simulink model "StampFly_KF400"  (R2026b)
settings: Solver=FixedStepDiscrete  StopTime=inf  FixedStep=Official.Step
PostLoadFcn:
  | run(fullfile(fileparts(get_param('StampFly_KF400','FileName')),'config','startup.m'));
InitFcn:
  | init_kf_flight;
undefined symbols (not defined in the file): AltitudeKF, Bottom, Discrete, Official, Time
libraries: slpidlib x7, simulink x4, ctrlSharedLib x1, mspfiltlib x1
(part 1 of 4)
settings Model: SILPILModeSetting=veronly  Creator=tyasukaw  LastModifiedBy=tyasukaw
settings SolverCC: AutoInsertRateTranBlk=on
settings OptimizationCC: DifferentSizesBufferReuse=on  EfficientTunableParamExpr=on  EnhancedBackFolding=on  MaxStackSize=64  OptimizationCustomize=off  OptimizeBlockOrder=speed  PassReuseOutputArgsAs=Individual arguments  RemoveInternalMemoryZeroInit=on  RemoveRootLevelIOMemoryZeroInit=on
settings DebuggingCC: ParameterTunabilityLossMsg=error
settings HardwareCC: ProdHWDeviceType=ARM Compatible->ARM Cortex  ProdLargestAtomicFloat=Double  ProdLargestAtomicInteger=Long
settings SFSimCC: MATLABDynamicMemAlloc=off
settings RTWCC: BuildConfiguration=Faster Runs  DataTypeReplacement=CDataTypesFixedWidth  Description=Embedded Coder  HardwareBoard=ESP32-S3 Series (Arduino Compatible)  SystemTargetFile=ert.tlc  TLCOptions="-aInlineSetEventsForThisBaseRateFcn=TLC_FALSE -aSuppressMultiTaskScheduler=TLC_FALSE  -aRateBasedStepFcn=0"  TemplateMakefile=ert_default_tmf  Toolchain=ESP32
settings CodeAppCC: ForceParamTrailComments=on  IgnoreCustomStorageClasses=off  InsertBlockDesc=on  OperatorAnnotations=on  SFDataObjDesc=on  SimulinkDataObjDesc=on
settings ERTTargetCC: CombineSignalStateStructs=on  ExtModeAutomaticAllocSize=off  ExtModeIntrfLevel=Level2 - Open  ExtModeMexFile=ext_xcp  ExtModeStaticAlloc=on  MaxIdInt16=INT16_MAX  MaxIdInt32=INT32_MAX  MaxIdInt64=INT64_MAX  MaxIdInt8=INT8_MAX  MaxIdUint16=UINT16_MAX  MaxIdUint32=UINT32_MAX  MaxIdUint64=UINT64_MAX  MaxIdUint8=UINT8_MAX  MinIdInt16=INT16_MIN  MinIdInt32=INT32_MIN  MinIdInt64=INT64_MIN  MinIdInt8=INT8_MIN  SupportContinuousTime=on  SupportVariableSizeSignals=on

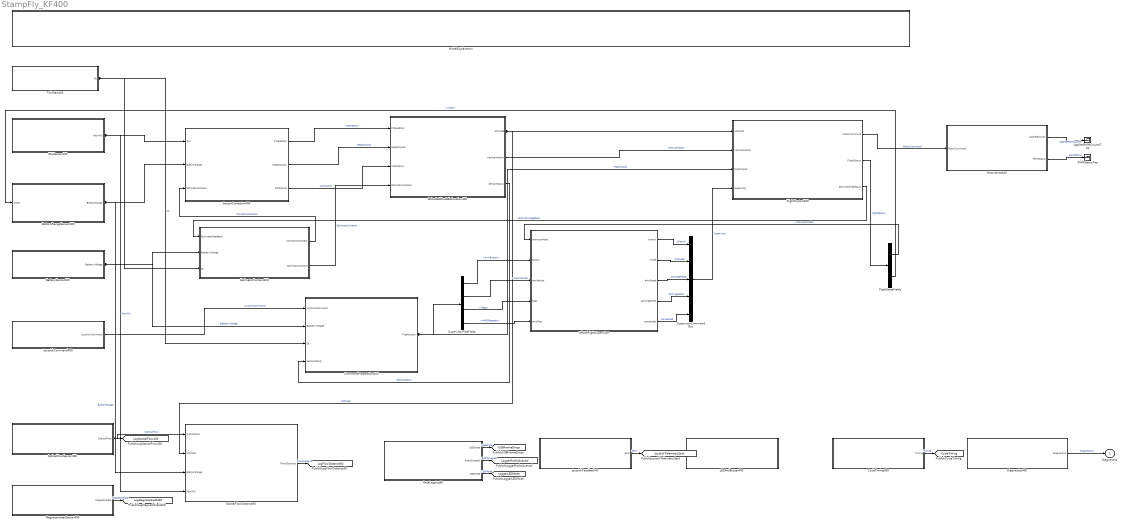
== system StampFly_KF400 ==
  AppliedPWMCountsTap : Terminator
  AttitudeAltitudeEstimation400 : Subsystem
      mask Display: disp('AttitudeAltitudeEstimation400');port_label('input',1,'FilteredIMU');port_label('input',2,'HeightInputs');port_label('input',3,'Calibration');port_label('input',4,'EstimatorContext');port_label('output',1,'Attitude');port_label('output',2,'VerticalMotion');port_label('output',3,'SensorStatus');
  BatterySensor400 : Subsystem
      mask Display: disp('BatterySensor400');port_label('output',1,'BatteryVoltage');
  BottomRangeSensor400 : Subsystem
      mask Display: disp('BottomRangeSensor400');port_label('input',1,'Mode');port_label('output',1,'BottomRange');
  CommandPreparation400 : Subsystem
      mask Display: disp('CommandPreparation400');port_label('input',1,'JoystickCommand');port_label('input',2,'BatteryVoltage');port_label('input',3,'Dt');port_label('input',4,'SensorStatus');port_label('output',1,'FlightInputs');
  CycleTiming400 : Subsystem
      mask Display: disp('CycleTiming400');port_label('output',1,'Timing');
  DataLogging50 : Subsystem
      mask Display: disp('DataLogging50');port_label('output',1,'USBDrops');port_label('output',2,'RadioQueued');port_label('output',3,'LEDMode');
  Diagnostics400 : Subsystem
      mask Display: disp('Diagnostics400');port_label('output',1,'Diagnostics');
  EstimatorContext400 : Subsystem
      mask Display: disp('EstimatorContext400');port_label('input',1,'EstimatorFeedback');port_label('input',2,'BatteryVoltage');port_label('input',3,'Dt');port_label('output',1,'CorrectionContext');port_label('output',2,'EstimatorContext');
  FlightControl400 : Subsystem
      mask Display: disp('FlightControl400');port_label('input',1,'Attitude');port_label('input',2,'VerticalMotion');port_label('input',3,'FlightInputs');port_label('input',4,'Supervisor');port_label('output',1,'MotorCommand');port_label('output',2,'FlightStatus');port_label('output',3,'EstimatorFeedback');
  FlightStateFields : BusSelector  OutputSignals=PreviousMode,Mode
  IMUSensor400 : Subsystem
      mask Display: disp('IMUSensor400');port_label('output',1,'RawIMU');
  JoystickCommand400 : Subsystem
      mask Display: disp('JoystickCommand400');port_label('output',1,'JoystickCommand');
  JoystickFeedback40 : Subsystem
      mask Display: disp('JoystickFeedback40');port_label('output',1,'Sent');
  LEDAndBuzzer400 : Subsystem
      mask Display: disp('LED・ブザー\n状態を表示')
  MagnetometerSensor400 : Subsystem
      mask Display: disp('MagnetometerSensor400');port_label('output',1,'MagneticField');
  ModelExplanation : Subsystem  Description=飛行成功版と等価性比較済み。学生が各機能を個別に編集できます。
      mask Display: disp(sprintf('StampFly IMU + Kalman Filter / 400 Hz\nセンサー取得 → 校正・前処理 → 標準の姿勢・高度推定 → PID → モーター\n飛行モードは最上位のStateflowで管理。下段は観測・記録・状態表示。'));
  MotorWrite400 : Subsystem
      mask Display: disp('MotorWrite400');port_label('input',1,'MotorCommand');port_label('output',1,'AppliedCounts');port_label('output',2,'PWMStatus');
  OfficialFlightSupervisor : Stateflow chart  Description=公式の待機・校正・飛行・着陸・通信断の状態遷移。Chart内部の状態と遷移は変更しない。  TreatAsAtomicUnit=on
  OpticalFlowDistance50 : Subsystem
      mask Display: disp('OpticalFlowDistance50');port_label('input',1,'OpticalFlow');port_label('input',2,'Attitude');port_label('input',3,'BottomRange');port_label('input',4,'RawIMU');port_label('output',1,'FlowDistance');
  OpticalFlowSensor400 : Subsystem
      mask Display: disp('OpticalFlowSensor400');port_label('output',1,'OpticalFlow');
  PWMStatusTap : Terminator
  SensorCorrection400 : Subsystem
      mask Display: disp('SensorCorrection400');port_label('input',1,'IMU');port_label('input',2,'BottomRange');port_label('input',3,'EstimatorContext');port_label('output',1,'FilteredIMU');port_label('output',2,'HeightInputs');port_label('output',3,'Calibration');
  SupervisorCommandBus : BusCreator  Inputs=5
  SupervisorPilotFields : BusSelector  OutputSignals=ArmButton,NewPacket,Flags,AHRSRequest
  TickStart400 : Subsystem
      mask Display: disp('TickStart400');port_label('output',1,'Dt');
  Diagnostics : Outport  OutDataTypeStr=Bus: OfficialDiagnosticBus  BusOutputAsStruct=on
  tag scope: CycleTiming=global, JoystickTelemetrySent=global, LogFlowDistance50=global, LogMagneticField400=global, LogOpticalFlow400=global, LoggerLEDMode=global, LoggerRadioQueued=global, USBFrameDrops=global
  wires:
  JoystickFeedback40/1(Sent) -> [JoystickTelemetrySent]  "Sent"
  CycleTiming400/1(Timing) -> [CycleTiming]  "Timing"
  AttitudeAltitudeEstimation400/2(VerticalMotion) -> FlightControl400/2(VerticalMotion)  "VerticalMotion"
  SensorCorrection400/1(FilteredIMU) -> AttitudeAltitudeEstimation400/1(FilteredIMU)  "FilteredIMU"
  SensorCorrection400/2(HeightInputs) -> AttitudeAltitudeEstimation400/2(HeightInputs)  "HeightInputs"
  SensorCorrection400/3(Calibration) -> AttitudeAltitudeEstimation400/3(Calibration)  "Calibration"
  Diagnostics400/1(Diagnostics) -> Diagnostics/1  "Diagnostics"
  DataLogging50/1(USBDrops) -> [USBFrameDrops]  "USBDrops"
  DataLogging50/2(RadioQueued) -> [LoggerRadioQueued]  "RadioQueued"
  DataLogging50/3(LEDMode) -> [LoggerLEDMode]  "LEDMode"
  SupervisorCommandBus/1 -> FlightControl400/4(Supervisor)  "Supervisor"
  OfficialFlightSupervisor/5(connected) -> SupervisorCommandBus/5  "Connected"
  OfficialFlightSupervisor/4(parkingReset) -> SupervisorCommandBus/4  "ParkingReset"
  OfficialFlightSupervisor/3(ahrsReset) -> SupervisorCommandBus/3  "AttitudeReset"
  OfficialFlightSupervisor/2(mode) -> SupervisorCommandBus/2  "PreMode"
  OfficialFlightSupervisor/1(branch) -> SupervisorCommandBus/1  "Branch"
  SupervisorPilotFields/4 -> OfficialFlightSupervisor/5(ahrsFlag)  "<AHRSRequest>"
  SupervisorPilotFields/3 -> OfficialFlightSupervisor/4(flags)  "<Flags>"
  SupervisorPilotFields/2 -> OfficialFlightSupervisor/3(newPacket)  "<NewPacket>"
  SupervisorPilotFields/1 -> OfficialFlightSupervisor/2(button)  "<ArmButton>"
  FlightStateFields/1 -> OfficialFlightSupervisor/1(previousMode)  "<PreviousMode>"
  FlightControl400/2(FlightStatus) -> FlightStateFields/1  "FlightStatus"
  FlightStateFields/2 -> BottomRangeSensor400/1(Mode)  "<Mode>"
  FlightControl400/1(MotorCommand) -> MotorWrite400/1(MotorCommand)  "MotorCommand"
  MotorWrite400/1(AppliedCounts) -> AppliedPWMCountsTap/1  "AppliedPWMCounts"
  MotorWrite400/2(PWMStatus) -> PWMStatusTap/1  "PWMStatus"
  AttitudeAltitudeEstimation400/3(SensorStatus) -> CommandPreparation400/4(SensorStatus)  "SensorStatus"
  CommandPreparation400/1(FlightInputs) -> SupervisorPilotFields/1, FlightControl400/3(FlightInputs)  "FlightInputs"
  TickStart400/1(Dt) -> EstimatorContext400/3(Dt), CommandPreparation400/3(Dt)  "Dt"
  BatterySensor400/1(BatteryVoltage) -> EstimatorContext400/2(BatteryVoltage), CommandPreparation400/2(BatteryVoltage)  "BatteryVoltage"
  JoystickCommand400/1(JoystickCommand) -> CommandPreparation400/1(JoystickCommand)  "JoystickCommand"
  EstimatorContext400/1(CorrectionContext) -> SensorCorrection400/3(EstimatorContext)  "CorrectionContext"
  FlightControl400/3(EstimatorFeedback) -> EstimatorContext400/1(EstimatorFeedback)  "EstimatorFeedback"
  EstimatorContext400/2(EstimatorContext) -> AttitudeAltitudeEstimation400/4(EstimatorContext)  "EstimatorContext"
  BottomRangeSensor400/1(BottomRange) -> SensorCorrection400/2(BottomRange), OpticalFlowDistance50/3(BottomRange)  "BottomRange"
  OpticalFlowSensor400/1(OpticalFlow) -> [LogOpticalFlow400], OpticalFlowDistance50/1(OpticalFlow)  "OpticalFlow"
  IMUSensor400/1(RawIMU) -> OpticalFlowDistance50/4(RawIMU), SensorCorrection400/1(IMU)  "RawIMU"
  AttitudeAltitudeEstimation400/1(Attitude) -> FlightControl400/1(Attitude), OpticalFlowDistance50/2(Attitude)  "Attitude"
  OpticalFlowDistance50/1(FlowDistance) -> [LogFlowDistance50]  "FlowDistance"
  MagnetometerSensor400/1(MagneticField) -> [LogMagneticField400]  "MagneticField"

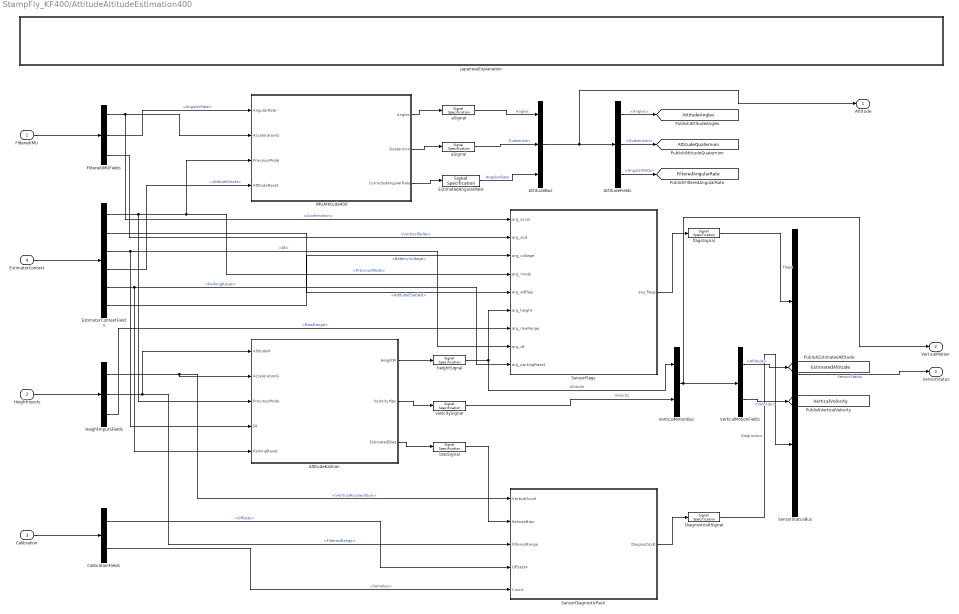
== system StampFly_KF400/AttitudeAltitudeEstimation400 ==
  FilteredIMU : Inport
  HeightInputs : Inport  Port=2
  Calibration : Inport  Port=3
  EstimatorContext : Inport  Port=4
  AltitudeKalman : Subsystem  Description=Standard time-varying altitude Kalman Filter. State [velocity;height;bias]. Current dt/az timing, original mode hold and private-state-retaining parking reset are preserved.  TreatAsAtomicUnit=on
  AttitudeBus : BusCreator  Inputs=3
  AttitudeFields : BusSelector  OutputSignals=Angles,Quaternion,AngularRate
  CalibrationFields : BusSelector  OutputSignals=Offsets,Samples
  Diagnostics8Signal : SignalSpecification  OutDataTypeStr=single  Dimensions=8
  EstimatedAngularRate : SignalSpecification  OutDataTypeStr=single  Dimensions=3
  EstimatorContextFields : BusSelector  OutputSignals=PreviousMode,AltitudeEnabled,Dt,AttitudeReset,ParkingReset,BatteryVoltage
  FilteredIMUFields : BusSelector  OutputSignals=Acceleration,AngularRate,VerticalDelta
  HeightInputsFields : BusSelector  OutputSignals=VerticalAcceleration,FilteredRange,RawRange
  IMUAttitude400 : Subsystem  Description=Standard IMU Filter: NED frame, 400 Hz, attitude and residual-bias-corrected gyro. Startup calibration, mode gating and flight conventions are retained.
  JapaneseExplanation : Subsystem  Description=|
      | 姿勢・高度推定 / 400 Hz
      | IMU Filterで姿勢・補正済み角速度、標準Kalman Filterで高度・鉛直速度を推定。
      | 加速度の単位・ToF前処理・PIDは飛行成功IMU版と共通。
      mask Display: disp(sprintf('姿勢・高度推定 / 400 Hz\nIMU Filterで姿勢・補正済み角速度、標準Kalman Filterで高度・鉛直速度を推定。\n加速度の単位・ToF前処理・PIDは飛行成功IMU版と共通。'));
  SensorDiagnosticPack : Subsystem  Description=記録用にまとめる
  SensorFlags : MATLAB Function  Description=距離異常・過加速度・低電圧  TreatAsAtomicUnit=on
  SensorStatusBus : BusCreator  Inputs=2
  VerticalMotionBus : BusCreator  Inputs=2
  VerticalMotionFields : BusSelector  OutputSignals=Altitude,Velocity
  aSignal : SignalSpecification  OutDataTypeStr=single  Dimensions=3
  biasSignal : SignalSpecification  OutDataTypeStr=single  Dimensions=1
  flagsSignal : SignalSpecification  OutDataTypeStr=uint8  Dimensions=3
  heightSignal : SignalSpecification  OutDataTypeStr=single  Dimensions=1
  qSignal : SignalSpecification  OutDataTypeStr=single  Dimensions=4
  velocitySignal : SignalSpecification  OutDataTypeStr=single  Dimensions=1
  Attitude : Outport
  VerticalMotion : Outport  Port=2
  SensorStatus : Outport  Port=3
  tag scope: AttitudeAngles=global, AttitudeQuaternion=global, EstimatedAltitude=global, FilteredAngularRate=global, VerticalVelocity=global
  wires:
  SensorDiagnosticPack/1(Diagnostics8) -> Diagnostics8Signal/1
  EstimatorContext/1 -> EstimatorContextFields/1
  HeightInputs/1 -> HeightInputsFields/1
  Calibration/1 -> CalibrationFields/1
  FilteredIMU/1 -> FilteredIMUFields/1
  EstimatorContextFields/6 -> SensorFlags/3(arg_voltage)  "<BatteryVoltage>"
  FilteredIMUFields/2 -> IMUAttitude400/1(AngularRate)  "<AngularRate>"
  EstimatorContextFields/2 -> SensorFlags/5(arg_altFlag)  "<AltitudeEnabled>"
  FilteredIMUFields/1 -> SensorFlags/1(arg_accel), IMUAttitude400/2(AccelerationG)  "<Acceleration>"
  FilteredIMUFields/3 -> SensorFlags/2(arg_azd)  "<VerticalDelta>"
  EstimatorContextFields/4 -> IMUAttitude400/4(AttitudeReset)  "<AttitudeReset>"
  IMUAttitude400/3(CorrectedAngularRate) -> EstimatedAngularRate/1
  HeightInputsFields/3 -> SensorFlags/7(arg_rawRange)  "<RawRange>"
  IMUAttitude400/1(Angles) -> aSignal/1
  IMUAttitude400/2(Quaternion) -> qSignal/1
  SensorFlags/1(arg_flags) -> flagsSignal/1
  aSignal/1 -> AttitudeBus/1  "Angles"
  AttitudeFields/1 -> [AttitudeAngles]  "<Angles>"
  EstimatedAngularRate/1 -> AttitudeBus/3  "AngularRate"
  qSignal/1 -> AttitudeBus/2  "Quaternion"
  VerticalMotionBus/1 -> VerticalMotionFields/1, VerticalMotion/1
  Diagnostics8Signal/1 -> SensorStatusBus/2  "Diagnostics"
  AttitudeFields/2 -> [AttitudeQuaternion]  "<Quaternion>"
  CalibrationFields/1 -> SensorDiagnosticPack/4(Offsets4)  "<Offsets>"
  AttitudeFields/3 -> [FilteredAngularRate]  "<AngularRate>"
  AttitudeBus/1 -> AttitudeFields/1, Attitude/1
  CalibrationFields/2 -> SensorDiagnosticPack/5(Count)  "<Samples>"
  flagsSignal/1 -> SensorStatusBus/1  "Flags"
  VerticalMotionFields/1 -> [EstimatedAltitude]  "<Altitude>"
  VerticalMotionFields/2 -> [VerticalVelocity]  "<Velocity>"
  SensorStatusBus/1 -> SensorStatus/1  "SensorStatus"
  AltitudeKalman/2(VelocityMps) -> velocitySignal/1
  AltitudeKalman/1(HeightM) -> heightSignal/1
  AltitudeKalman/3(EstimatedBias) -> biasSignal/1
  biasSignal/1 -> SensorDiagnosticPack/2(KalmanBias)
  velocitySignal/1 -> VerticalMotionBus/2  "Velocity"
  heightSignal/1 -> VerticalMotionBus/1, SensorFlags/6(arg_height)  "Altitude"
  EstimatorContextFields/3 -> AltitudeKalman/4(Dt), SensorFlags/8(arg_dt)  "<Dt>"
  HeightInputsFields/2 -> AltitudeKalman/1(AltitudeM), SensorDiagnosticPack/3(FilteredRange)  "<FilteredRange>"
  EstimatorContextFields/1 -> IMUAttitude400/3(PreviousMode), SensorFlags/4(arg_mode), AltitudeKalman/3(PreviousMode)  "<PreviousMode>"
  EstimatorContextFields/5 -> SensorFlags/9(arg_parkingReset), AltitudeKalman/5(ParkingReset)  "<ParkingReset>"
  HeightInputsFields/1 -> AltitudeKalman/2(AccelerationG), SensorDiagnosticPack/1(VerticalAccel)  "<VerticalAcceleration>"

== system StampFly_KF400/BatterySensor400 ==
  Battery400 : MATLABSystem  Description=電池電圧：I2C読出しはcore0。400 Hz側は最新値と100 ms以内の有効性を返し、待たない。  Priority=4  System=official.Battery400  SampleTime=Official.Step  SimulateUsing=Code generation
      mask Type: official.Battery400
  BatteryVoltage : Outport
  tag scope: BatteryReadValid=global, BatteryVoltage=global
  wires:
  Battery400/2 -> [BatteryReadValid]  "BatteryValid"
  Battery400/1 -> BatteryVoltage/1, [BatteryVoltage]  "BatteryVoltage"

== system StampFly_KF400/BottomRangeSensor400 ==
  Mode : Inport
  BottomRangeFields : BusSelector  OutputSignals=DistanceMm,Fresh
  BottomToF400 : Subsystem
  JapaneseExplanation : Subsystem  Description=|
      | 下向きToFの取得
      | VL53L3CXは測定準備完了時に読み出し、400 Hz側では最新値を保持します。
      | BottomRange = DistanceMm[int16] + Fresh[uint8]。元の前周期モード参照も保持。
      | 前向きToFは無効。Optical Flowは未実装。
      mask Display: disp('下向きToFの取得\nVL53L3CXは測定準備完了時に読み出し、400 Hz側では最新値を保持します。\nBottomRange = DistanceMm[int16] + Fresh[uint8]。元の前周期モード参照も保持。\n前向きToFは無効。Optical Flowは未実装。')
  RangeDiagnosticsFields : BusSelector  OutputSignals=FrontDistanceMm,Status,Info
  BottomRange : Outport
  tag scope: BottomDistanceMm=global, BottomRangeFresh=global, BottomRangeStatus=global, BottomToFDiagnostics=global, UnusedFrontRangeMm=global
  wires:
  Mode/1 -> BottomToF400/1(FinalMode)
  BottomRangeFields/2 -> [BottomRangeFresh]  "<Fresh>"
  BottomRangeFields/1 -> [BottomDistanceMm]  "<DistanceMm>"
  BottomToF400/2(RangeDiagnostics) -> RangeDiagnosticsFields/1  "RangeDiagnostics"
  BottomToF400/1(BottomRange) -> BottomRange/1, BottomRangeFields/1  "BottomRange"
  RangeDiagnosticsFields/3 -> [BottomToFDiagnostics]  "<Info>"
  RangeDiagnosticsFields/2 -> [BottomRangeStatus]  "<Status>"
  RangeDiagnosticsFields/1 -> [UnusedFrontRangeMm]  "<FrontDistanceMm>"

== system StampFly_KF400/CommandPreparation400 ==
  JoystickCommand : Inport
  BatteryVoltage : Inport  Port=2
  Dt : Inport  Port=3
  SensorStatus : Inport  Port=4
  CommandTapFields : BusSelector  OutputSignals=Sticks,AHRSRequest
  FlightInputBus400 : Subsystem
  JapaneseExplanation : Subsystem  Description=|
      | 操作入力をFlightInputsバスへまとめます。
      | JoyStickの操作、電池電圧、実測Dt、推定系のSensorStatusを直接接続。
      | この部分は信号の整理だけで、制御則や遅延を追加しません。
      mask Display: disp('操作入力をFlightInputsバスへまとめます。\nJoyStickの操作、電池電圧、実測Dt、推定系のSensorStatusを直接接続。\nこの部分は信号の整理だけで、制御則や遅延を追加しません。')
  SensorTapFields : BusSelector  OutputSignals=Flags,Diagnostics
  FlightInputs : Outport
  tag scope: AttitudeResetRequest=global, JoystickSticks=global, SensorDiagnostics=global, SensorFlags=global
  wires:
  FlightInputBus400/2(CommandTap) -> CommandTapFields/1  "CommandTap"
  CommandTapFields/1 -> [JoystickSticks]  "<Sticks>"
  CommandTapFields/2 -> [AttitudeResetRequest]  "<AHRSRequest>"
  BatteryVoltage/1 -> FlightInputBus400/2(BatteryVoltage)
  FlightInputBus400/3(SensorTap) -> SensorTapFields/1  "SensorTap"
  JoystickCommand/1 -> FlightInputBus400/1(JoystickCommand)
  FlightInputBus400/1(FlightInputs) -> FlightInputs/1  "FlightInputs"
  SensorStatus/1 -> FlightInputBus400/4(SensorStatus)
  Dt/1 -> FlightInputBus400/3(Dt)
  SensorTapFields/1 -> [SensorFlags]  "<Flags>"
  SensorTapFields/2 -> [SensorDiagnostics]  "<Diagnostics>"

== system StampFly_KF400/CycleTiming400 ==
  TimingEnd400 : MATLABSystem  Description=処理時間測定：周期開始からこのブロックまでの時間を測ります。平均・最大・開始間隔・超過回数を取得します。  Priority=10000  System=official.TimingEnd400  SampleTime=Official.Step  SimulateUsing=Code generation
      mask Type: official.TimingEnd400
  Timing : Outport
  wires:
  [PWMStatus] -> TimingEnd400/4
  [AppliedPWMCounts] -> TimingEnd400/3
  [IMUSampleFresh] -> TimingEnd400/2
  [CycleStartUs] -> TimingEnd400/1
  TimingEnd400/1 -> Timing/1  "Timing"
  [USBFrameDrops] -> TimingEnd400/5

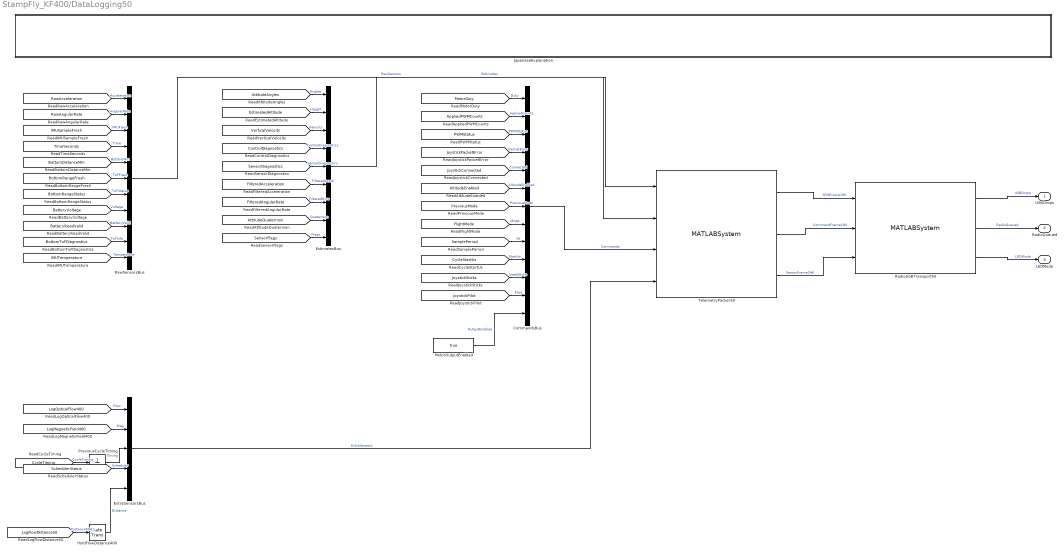
== system StampFly_KF400/DataLogging50 ==
  CommandsBus : BusCreator  Inputs=13  OutDataTypeStr=Bus: BasicLogCommandBus  NonVirtualBus=on
  EstimatesBus : BusCreator  Inputs=9  OutDataTypeStr=Bus: LogEstimateBus  NonVirtualBus=on
  ExtraSensorsBus : BusCreator  Inputs=5  OutDataTypeStr=Bus: LogExtraBus  NonVirtualBus=on
  HoldFlowDistance400 : RateTransition  OutPortSampleTime=.0025
  JapaneseExplanation : Subsystem  Description=|
      | 記録（50 Hz）
      | 元のstampfly_imu_monitor由来のSFI8パケットとMATロガーを継続使用。
      | 下向きToF・姿勢・高度・Duty・制御診断を保存。Optical Flowは未実装のためNaN。
      mask Display: disp(sprintf('データ記録 / 50 Hz\n磁気・光学フロー・ToF・推定・制御を名前付きFromから取得。\nSFI8 / SFIX / SFIYのパケット形式を維持。'));
  MotorOutputEnabled : Constant  Value=true  OutDataTypeStr=boolean
  PreviousCycleTiming : UnitDelay  InitialCondition=zeros(8,1,'uint32')  SampleTime=.0025
  RadioUSBTransport50 : MATLABSystem  System=official.LogTransport50  SimulateUsing=Code generation
      mask Type: official.LogTransport50
  RawSensorsBus : BusCreator  Inputs=11  OutDataTypeStr=Bus: LogRawBus  NonVirtualBus=on
  TelemetryPacker50 : MATLABSystem  System=basic.ExtendedLogger50  BuildID=uint32( 1401 )  FirmwareRevision=uint32(1801)  SimulateUsing=Code generation
      mask Type: basic.ExtendedLogger50
  USBDrops : Outport
  RadioQueued : Outport  Port=2
  LEDMode : Outport  Port=3
  wires:
  [SamplePeriod] -> CommandsBus/9  "Dt"
  [FilteredAngularRate] -> EstimatesBus/7  "FilteredGyro"
  [LogFlowDistance50] -> HoldFlowDistance400/1  "Distance50Hz"
  [BottomRangeFresh] -> RawSensorsBus/6  "ToFFresh"
  [CycleStartUs] -> CommandsBus/10  "StartUs"
  [JoystickConnected] -> CommandsBus/5  "Connected"
  [PWMStatus] -> CommandsBus/3  "PWMStatus"
  [TimeSeconds] -> RawSensorsBus/4  "Time"
  [LogOpticalFlow400] -> ExtraSensorsBus/1  "Flow"
  [SensorDiagnostics] -> EstimatesBus/5  "SensorDiagnostics"
  [BottomToFDiagnostics] -> RawSensorsBus/10  "ToFInfo"
  [IMUSampleFresh] -> RawSensorsBus/3  "IMUFresh"
  [JoystickSticks] -> CommandsBus/11  "UsedSticks"
  [FilteredAcceleration] -> EstimatesBus/6  "FilteredAccel"
  [RawAngularRate] -> RawSensorsBus/2  "AngularRate"
  [JoystickPilot] -> CommandsBus/12  "Pilot"
  [EstimatedAltitude] -> EstimatesBus/2  "Height"
  [RawAcceleration] -> RawSensorsBus/1  "Acceleration"
  [PreviousMode] -> CommandsBus/7  "PreviousMode"
  [JoystickPacketError] -> CommandsBus/4  "PacketError"
  [VerticalVelocity] -> EstimatesBus/3  "Velocity"
  [CycleTiming] -> PreviousCycleTiming/1  "CycleTiming"
  [BottomDistanceMm] -> RawSensorsBus/5  "BottomMm"
  [SchedulerStatus] -> ExtraSensorsBus/4  "Scheduler"
  [LogMagneticField400] -> ExtraSensorsBus/2  "Mag"
  [FlightMode] -> CommandsBus/8  "Mode"
  [BottomRangeStatus] -> RawSensorsBus/7  "ToFStatus"
  PreviousCycleTiming/1 -> ExtraSensorsBus/3  "Timing"
  [BatteryVoltage] -> RawSensorsBus/8  "Voltage"
  [BatteryReadValid] -> RawSensorsBus/9  "BatteryValid"
  [MotorDuty] -> CommandsBus/1  "Duty"
  [SensorFlags] -> EstimatesBus/9  "Flags"
  [ControlDiagnostics] -> EstimatesBus/4  "ControlDiagnostics"
  [IMUTemperature] -> RawSensorsBus/11  "Temperature"
  HoldFlowDistance400/1 -> ExtraSensorsBus/5  "Distance"
  [AttitudeAngles] -> EstimatesBus/1  "Angles"
  [AttitudeQuaternion] -> EstimatesBus/8  "Quaternion"
  [AppliedPWMCounts] -> CommandsBus/2  "AppliedCounts"
  RadioUSBTransport50/2 -> RadioQueued/1  "RadioQueued"
  ExtraSensorsBus/1 -> TelemetryPacker50/4  "ExtraSensors"
  [AltitudeEnabled] -> CommandsBus/6  "AltitudeEnabled"
  RawSensorsBus/1 -> TelemetryPacker50/1  "RawSensors"
  MotorOutputEnabled/1 -> CommandsBus/13  "OutputEnabled"
  EstimatesBus/1 -> TelemetryPacker50/2  "Estimates"
  CommandsBus/1 -> TelemetryPacker50/3  "Commands"
  TelemetryPacker50/1 -> RadioUSBTransport50/1  "SFI8Frame190"
  TelemetryPacker50/2 -> RadioUSBTransport50/2  "CommandFrame190"
  TelemetryPacker50/3 -> RadioUSBTransport50/3  "SensorFrame246"
  RadioUSBTransport50/1 -> USBDrops/1  "USBDrops"
  RadioUSBTransport50/3 -> LEDMode/1  "LEDMode"

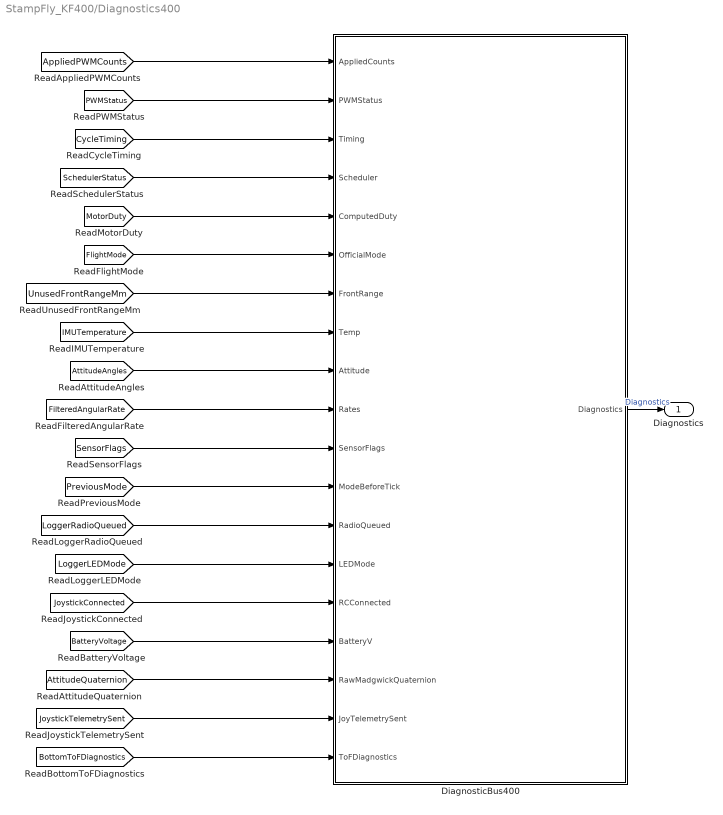
== system StampFly_KF400/Diagnostics400 ==
  DiagnosticBus400 : Subsystem
      mask Display: disp('DiagnosticBus400');port_label('input',1,'AppliedCounts');port_label('input',2,'PWMStatus');port_label('input',3,'Timing');port_label('input',4,'Scheduler');port_label('input',5,'ComputedDuty');port_label('input',6,'OfficialMode');port_label('input',7,'FrontRange');port_label('input',8,'Temp');port_label('input',9,'Attitude');port_label('input',10,'Rates');port_label('input',11,'SensorFlags');port_label('input',12,'ModeBeforeTick');port_label('input',13,'RadioQueued');port_label('input',14,'LEDMode');port_label('input',15,'RCConnected');port_label('input',16,'BatteryV');port_label('input',17,'RawMadgwickQuaternion');port_label('input',18,'JoyTelemetrySent');port_label('input',19,'ToFDiagnostics');port_label('output',1,'Diagnostics');
  Diagnostics : Outport
  wires:
  [FlightMode] -> DiagnosticBus400/6(OfficialMode)
  [CycleTiming] -> DiagnosticBus400/3(Timing)
  [BottomToFDiagnostics] -> DiagnosticBus400/19(ToFDiagnostics)
  [AppliedPWMCounts] -> DiagnosticBus400/1(AppliedCounts)
  [SchedulerStatus] -> DiagnosticBus400/4(Scheduler)
  [IMUTemperature] -> DiagnosticBus400/8(Temp)
  [JoystickTelemetrySent] -> DiagnosticBus400/18(JoyTelemetrySent)
  [UnusedFrontRangeMm] -> DiagnosticBus400/7(FrontRange)
  [MotorDuty] -> DiagnosticBus400/5(ComputedDuty)
  [PWMStatus] -> DiagnosticBus400/2(PWMStatus)
  [AttitudeAngles] -> DiagnosticBus400/9(Attitude)
  [FilteredAngularRate] -> DiagnosticBus400/10(Rates)
  [JoystickConnected] -> DiagnosticBus400/15(RCConnected)
  [SensorFlags] -> DiagnosticBus400/11(SensorFlags)
  [PreviousMode] -> DiagnosticBus400/12(ModeBeforeTick)
  [LoggerRadioQueued] -> DiagnosticBus400/13(RadioQueued)
  [LoggerLEDMode] -> DiagnosticBus400/14(LEDMode)
  [BatteryVoltage] -> DiagnosticBus400/16(BatteryV)
  [AttitudeQuaternion] -> DiagnosticBus400/17(RawMadgwickQuaternion)
  DiagnosticBus400/1(Diagnostics) -> Diagnostics/1  "Diagnostics"

== system StampFly_KF400/EstimatorContext400 ==
  EstimatorFeedback : Inport
  BatteryVoltage : Inport  Port=2
  Dt : Inport  Port=3
  CorrectionContextInternal : BusCreator  Inputs=2
  EstimatorContextInternal : BusCreator  Inputs=6
  EstimatorFeedbackFields : BusSelector  OutputSignals=PreviousMode,AltitudeEnabled,AttitudeReset,ParkingReset
  JapaneseExplanation : Subsystem  Description=|
      | 推定系へのフィードバック配線
      | モード・高度制御フラグ・姿勢／待機リセットを意味のあるBusに整理。
      | 元の遅延はFlightControl400内に保持。この配線ブロック自体には新しい遅延を追加しません。
      mask Display: disp('推定系へのフィードバック配線\nモード・高度制御フラグ・姿勢／待機リセットを意味のあるBusに整理。\n元の遅延はFlightControl400内に保持。この配線ブロック自体には新しい遅延を追加しません。')
  CorrectionContext : Outport
  EstimatorContext : Outport  Port=2
  wires:
  CorrectionContextInternal/1 -> CorrectionContext/1  "CorrectionContext"
  BatteryVoltage/1 -> EstimatorContextInternal/6
  Dt/1 -> EstimatorContextInternal/3, CorrectionContextInternal/2
  EstimatorFeedback/1 -> EstimatorFeedbackFields/1
  EstimatorFeedbackFields/3 -> EstimatorContextInternal/4  "<AttitudeReset>"
  EstimatorFeedbackFields/1 -> CorrectionContextInternal/1, EstimatorContextInternal/1  "<PreviousMode>"
  EstimatorFeedbackFields/4 -> EstimatorContextInternal/5  "<ParkingReset>"
  EstimatorFeedbackFields/2 -> EstimatorContextInternal/2  "<AltitudeEnabled>"
  EstimatorContextInternal/1 -> EstimatorContext/1  "EstimatorContext"

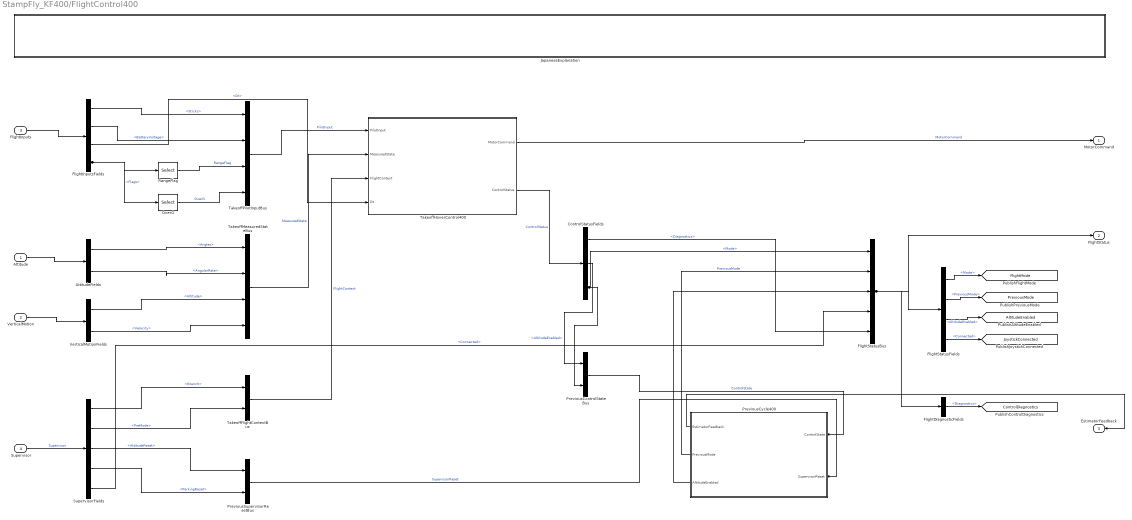
== system StampFly_KF400/FlightControl400 ==
  Attitude : Inport
  VerticalMotion : Inport  Port=2
  FlightInputs : Inport  Port=3
  Supervisor : Inport  Port=4
  AttitudeFields : BusSelector  OutputSignals=Angles,AngularRate
  ControlStatusFields : BusSelector  OutputSignals=Diagnostics,AltitudeEnabled,Mode
  FlightDiagnosticFields : BusSelector  OutputSignals=Diagnostics
  FlightInputsFields : BusSelector  OutputSignals=Sticks,BatteryVoltage,Dt,Flags
  FlightStatusBus : BusCreator  Inputs=5
  FlightStatusFields : BusSelector  OutputSignals=Mode,PreviousMode,AltitudeEnabled,Connected
  JapaneseExplanation : Subsystem  Description=|
      | 飛行制御：400 Hz（2.5 ms）
      | 推定値・操作入力 → Stateflowの飛行モード → 離陸・ホバリング制御 → モーター指令。
      | 下段は元の1周期遅延。推定器とモード判断へ直接戻します。ロガー・通信の形式は維持しています。
      mask Display: disp(sprintf('飛行制御 / 400 Hz\n最上位Stateflowの指令 → 離着陸・7個のPID → モーター指令\n前周期の保持と飛行状態ログはこの内部。'));
  OverG : Selector  InputPortWidth=3  IndexOptions=Index vector (dialog)  Indices=1  OutputSizes=1
  PreviousControlStateBus : BusCreator  Inputs=2
  PreviousCycle400 : Subsystem  Description=元のUnit Delayと型変換を保持する。モード・リセット・角速度指令などを元と同じ1周期遅延で返す。
      mask Display: disp('PreviousCycle400');port_label('input',1,'ControlState');port_label('input',2,'SupervisorReset');port_label('output',1,'EstimatorFeedback');port_label('output',2,'PreviousMode');port_label('output',3,'AltitudeEnabled');
  PreviousSupervisorResetBus : BusCreator  Inputs=2
  RangeFlag : Selector  InputPortWidth=3  IndexOptions=Index vector (dialog)  Indices=2  OutputSizes=1
  SupervisorFields : BusSelector  OutputSignals=Branch,PreMode,AttitudeReset,ParkingReset,Connected
  TakeoffFlightContextBus : BusCreator  Inputs=2
  TakeoffHoverControl400 : Subsystem  Description=離陸・着陸指令、高度・姿勢角・角速度のPID、モーター配分を機能別のブロックで構成する。
      mask Display: disp('TakeoffHoverControl400');port_label('input',1,'PilotInput');port_label('input',2,'MeasuredState');port_label('input',3,'FlightContext');port_label('input',4,'Dt');port_label('output',1,'MotorCommand');port_label('output',2,'ControlStatus');
  TakeoffMeasuredStateBus : BusCreator  Inputs=4
  TakeoffPilotInputBus : BusCreator  Inputs=4
  VerticalMotionFields : BusSelector  OutputSignals=Altitude,Velocity
  MotorCommand : Outport
  FlightStatus : Outport  Port=2
  EstimatorFeedback : Outport  Port=3
  tag scope: AltitudeEnabled=global, ControlDiagnostics=global, FlightMode=global, JoystickConnected=global, PreviousMode=global
  wires:
  FlightInputsFields/2 -> TakeoffPilotInputBus/2  "<BatteryVoltage>"
  Supervisor/1 -> SupervisorFields/1  "Supervisor"
  FlightDiagnosticFields/1 -> [ControlDiagnostics]  "<Diagnostics>"
  VerticalMotion/1 -> VerticalMotionFields/1
  Attitude/1 -> AttitudeFields/1
  TakeoffPilotInputBus/1 -> TakeoffHoverControl400/1(PilotInput)  "PilotInput"
  FlightInputsFields/4 -> OverG/1, RangeFlag/1  "<Flags>"
  FlightInputs/1 -> FlightInputsFields/1
  FlightInputsFields/3 -> TakeoffHoverControl400/4(Dt)  "<Dt>"
  FlightInputsFields/1 -> TakeoffPilotInputBus/1  "<Sticks>"
  RangeFlag/1 -> TakeoffPilotInputBus/3  "RangeFlag"
  OverG/1 -> TakeoffPilotInputBus/4  "OverG"
  AttitudeFields/1 -> TakeoffMeasuredStateBus/1  "<Angles>"
  AttitudeFields/2 -> TakeoffMeasuredStateBus/2  "<AngularRate>"
  VerticalMotionFields/1 -> TakeoffMeasuredStateBus/3  "<Altitude>"
  ControlStatusFields/2 -> PreviousControlStateBus/1  "<AltitudeEnabled>"
  VerticalMotionFields/2 -> TakeoffMeasuredStateBus/4  "<Velocity>"
  SupervisorFields/1 -> TakeoffFlightContextBus/1  "<Branch>"
  SupervisorFields/2 -> TakeoffFlightContextBus/2  "<PreMode>"
  PreviousSupervisorResetBus/1 -> PreviousCycle400/2(SupervisorReset)  "SupervisorReset"
  SupervisorFields/3 -> PreviousSupervisorResetBus/1  "<AttitudeReset>"
  SupervisorFields/4 -> PreviousSupervisorResetBus/2  "<ParkingReset>"
  SupervisorFields/5 -> FlightStatusBus/4  "<Connected>"
  TakeoffMeasuredStateBus/1 -> TakeoffHoverControl400/2(MeasuredState)  "MeasuredState"
  TakeoffFlightContextBus/1 -> TakeoffHoverControl400/3(FlightContext)  "FlightContext"
  TakeoffHoverControl400/1(MotorCommand) -> MotorCommand/1  "MotorCommand"
  TakeoffHoverControl400/2(ControlStatus) -> ControlStatusFields/1  "ControlStatus"
  ControlStatusFields/1 -> FlightStatusBus/5  "<Diagnostics>"
  ControlStatusFields/3 -> FlightStatusBus/1, PreviousControlStateBus/2  "<Mode>"
  FlightStatusBus/1 -> FlightDiagnosticFields/1, FlightStatusFields/1, FlightStatus/1
  FlightStatusFields/2 -> [PreviousMode]  "<PreviousMode>"
  PreviousCycle400/3(AltitudeEnabled) -> FlightStatusBus/3
  FlightStatusFields/1 -> [FlightMode]  "<Mode>"
  PreviousCycle400/2(PreviousMode) -> FlightStatusBus/2  "PreviousMode"
  PreviousCycle400/1(EstimatorFeedback) -> EstimatorFeedback/1
  FlightStatusFields/3 -> [AltitudeEnabled]  "<AltitudeEnabled>"
  FlightStatusFields/4 -> [JoystickConnected]  "<Connected>"
  PreviousControlStateBus/1 -> PreviousCycle400/1(ControlState)  "ControlState"

== system StampFly_KF400/IMUSensor400 ==
  BMI270_400 : MATLABSystem  Description=BMI270取得：加速度[m/s²]・角速度[rad/s]・温度・新規データ有無。センサーODRは400 Hzです。  Priority=2  System=stampfly.BMI270IMU  SampleTime=Official.Step  SimulateUsing=Code generation
      mask Type: stampfly.BMI270IMU
  JapaneseExplanation : Subsystem  Description=|
      | BMI270から加速度[m/s^2]・角速度[rad/s]を400 Hzで取得。
      | RawIMUの2要素を補正へ直接渡します。温度[degC]・Freshは記録用タグへ。
      | 温度はセンサー内部で約10 Hz更新。低レベルのSPI処理は専用Systemブロックが担当。
      mask Display: disp('BMI270から加速度[m/s^2]・角速度[rad/s]を400 Hzで取得。\nRawIMUの2要素を補正へ直接渡します。温度[degC]・Freshは記録用タグへ。\n温度はセンサー内部で約10 Hz更新。低レベルのSPI処理は専用Systemブロックが担当。')
  RawIMUInternal : BusCreator  Inputs=2
  RawIMU : Outport
  tag scope: IMUSampleFresh=global, IMUTemperature=global, RawAcceleration=global, RawAngularRate=global
  wires:
  BMI270_400/1 -> RawIMUInternal/1, [RawAcceleration]  "Acceleration"
  BMI270_400/2 -> RawIMUInternal/2, [RawAngularRate]  "AngularRate"
  RawIMUInternal/1 -> RawIMU/1  "RawIMU"
  BMI270_400/3 -> [IMUTemperature]  "Temperature"
  BMI270_400/4 -> [IMUSampleFresh]  "IMUFresh"

== system StampFly_KF400/JoystickCommand400 ==
  JoyStickInput400 : Subsystem
  RadioDiagnosticsFields : BusSelector  OutputSignals=LinkAge,PacketError
  RawRadioAgeUnused : Terminator
  JoystickCommand : Outport
  tag scope: JoystickPacketError=global, JoystickPilot=global
  wires:
  JoyStickInput400/1(JoystickCommand) -> [JoystickPilot], JoystickCommand/1  "JoystickCommand"
  RadioDiagnosticsFields/1 -> RawRadioAgeUnused/1  "<LinkAge>"
  JoyStickInput400/2(RadioDiagnostics) -> RadioDiagnosticsFields/1  "RadioDiagnostics"
  RadioDiagnosticsFields/2 -> [JoystickPacketError]  "<PacketError>"

== system StampFly_KF400/JoystickFeedback40 ==
  JapaneseExplanation : Subsystem  Description=公式JoyStickへ40 Hzで姿勢・高度・電圧・指令値を返信します。バイト形式は初回飛行版と同じ。
      mask Display: disp('公式JoyStickへ40 Hzで姿勢・高度・電圧・指令値を返信します。バイト形式は初回飛行版と同じ。')
  JoyStickTelemetry40 : Subsystem  Description=公式JoyStickへ40 Hzで姿勢・高度・電圧等を返信。前向きToFは無効で0を返信。
      mask Display: disp('JoyStickTelemetry40');port_label('input',1,'AltFlag');port_label('input',2,'Mode');port_label('input',3,'FrontMm');port_label('input',4,'TimeSec');port_label('input',5,'Dt');port_label('input',6,'Attitude3');port_label('input',7,'Rates3');port_label('input',8,'ControlDiag17');port_label('input',9,'Accel3');port_label('input',10,'BatteryV');port_label('input',11,'Duty4');port_label('input',12,'Height');port_label('input',13,'SensorDiag8');port_label('input',14,'Velocity');port_label('output',1,'Sent');
  Sent : Outport
  wires:
  [FlightMode] -> JoyStickTelemetry40/2(Mode)
  [EstimatedAltitude] -> JoyStickTelemetry40/12(Height)
  [AltitudeEnabled] -> JoyStickTelemetry40/1(AltFlag)
  [UnusedFrontRangeMm] -> JoyStickTelemetry40/3(FrontMm)
  [SamplePeriod] -> JoyStickTelemetry40/5(Dt)
  [TimeSeconds] -> JoyStickTelemetry40/4(TimeSec)
  [ControlDiagnostics] -> JoyStickTelemetry40/8(ControlDiag17)
  [FilteredAngularRate] -> JoyStickTelemetry40/7(Rates3)
  [AttitudeAngles] -> JoyStickTelemetry40/6(Attitude3)
  [RawAcceleration] -> JoyStickTelemetry40/9(Accel3)
  [BatteryVoltage] -> JoyStickTelemetry40/10(BatteryV)
  JoyStickTelemetry40/1(Sent) -> Sent/1  "Sent"
  [MotorDuty] -> JoyStickTelemetry40/11(Duty4)
  [SensorDiagnostics] -> JoyStickTelemetry40/13(SensorDiag8)
  [VerticalVelocity] -> JoyStickTelemetry40/14(Velocity)

== system StampFly_KF400/LEDAndBuzzer400 ==
  StatusOutputs400 : Subsystem  Description=LED・ブザー・ボタン｜表示判断はモデル、出力はドライバー
      mask Display: disp('StatusOutputs400');port_label('input',1,'Stick6');port_label('input',2,'SensorFlags3');port_label('input',3,'ModeBeforeTick');port_label('input',4,'AltFlag');port_label('input',5,'PacketError');port_label('input',6,'AHRSFlag');
  wires:
  [AttitudeResetRequest] -> StatusOutputs400/6(AHRSFlag)
  [SensorFlags] -> StatusOutputs400/2(SensorFlags3)
  [JoystickSticks] -> StatusOutputs400/1(Stick6)
  [JoystickPacketError] -> StatusOutputs400/5(PacketError)
  [AltitudeEnabled] -> StatusOutputs400/4(AltFlag)
  [PreviousMode] -> StatusOutputs400/3(ModeBeforeTick)

== system StampFly_KF400/MagnetometerSensor400 ==
  DeviceRead : MATLABSystem  System=stampfly.BMM150  I2CAddress=uint8( 16 )  SampleTime=.0025  SimulateUsing=Code generation
      mask Type: stampfly.BMM150
  JapaneseExplanation : Subsystem  Description=磁気取得専用：BMM150の新規測定30 Hz。400 Hz側はcore0の最新値を非待機で受け取ります。
      mask Display: disp('磁気取得専用：BMM150の新規測定30 Hz。400 Hz側はcore0の最新値を非待機で受け取ります。')
  SensorDataBus : BusCreator  Inputs=3  OutDataTypeStr=Bus: LogMagBus  NonVirtualBus=on
  MagneticField : Outport
  wires:
  SensorDataBus/1 -> MagneticField/1  "SensorData"
  DeviceRead/1 -> SensorDataBus/1  "Field"
  DeviceRead/2 -> SensorDataBus/2  "Flags"
  DeviceRead/3 -> SensorDataBus/3  "Info"

== system StampFly_KF400/ModelExplanation ==

== system StampFly_KF400/MotorWrite400 ==
  MotorCommand : Inport
  JapaneseExplanation : Subsystem  Description=|
      | モーターへの書込み
      | MotorCommand = Duty[4x1 single] + Counts[4x1 uint8]。順序は FR / FL / RR / RL。
      | LEDCへ400 HzでDuty指令を更新。キャリア150 kHz指定、8 bit。Duty上限0.95は制御側で保持。
      | 実際に適用されたCountsとPWM診断は記録用タグにも出力します。
      mask Display: disp('モーターへの書込み\nMotorCommand = Duty[4x1 single] + Counts[4x1 uint8]。順序は FR / FL / RR / RL。\nLEDCへ400 HzでDuty指令を更新。キャリア150 kHz指定、8 bit。Duty上限0.95は制御側で保持。\n実際に適用されたCountsとPWM診断は記録用タグにも出力します。')
  MotorCommandFields : BusSelector  OutputSignals=Duty,Counts
  MotorOutputs400 : Subsystem  Description=モーター出力｜400 Hz更新・150 kHz／8 bit
      mask Display: disp('MotorOutputs400');port_label('input',1,'Counts4');port_label('output',1,'AppliedCounts4');port_label('output',2,'PWMInfo4');
  AppliedCounts : Outport
  PWMStatus : Outport  Port=2
  tag scope: AppliedPWMCounts=global, MotorDuty=global, PWMStatus=global
  wires:
  MotorOutputs400/1(AppliedCounts4) -> AppliedCounts/1, [AppliedPWMCounts]  "AppliedCounts"
  MotorCommandFields/1 -> [MotorDuty]  "<Duty>"
  MotorCommand/1 -> MotorCommandFields/1
  MotorOutputs400/2(PWMInfo4) -> PWMStatus/1, [PWMStatus]  "PWMStatus"
  MotorCommandFields/2 -> MotorOutputs400/1(Counts4)  "<Counts>"

== system StampFly_KF400/OpticalFlowDistance50 ==
  OpticalFlow : Inport
  Attitude : Inport  Port=2
  BottomRange : Inport  Port=3
  RawIMU : Inport  Port=4
  AttitudeFields : BusSelector  OutputSignals=Angles
  DistanceData : BusCreator  Inputs=3  OutDataTypeStr=Bus: LogDistanceBus  NonVirtualBus=on
  FlowFields : BusSelector  OutputSignals=Totals,Raw
  GroundMotionDistance : MATLABSystem  System=imu.FlowDistance50  SampleTime=0.02  XCountsPerRad=385  YCountsPerRad=385  MinQuality=25  MaxHeightM=2  MaxHorizontalSpeedMps=1.5  MaxVerticalSpeedMps=2  MinDownProjection=0.5  SimulateUsing=Code generation
      mask Type: imu.FlowDistance50
  IMUFields : BusSelector  OutputSignals=AngularRate
  JapaneseExplanation : Subsystem  Description=移動距離への換算（表示・記録専用）\n400 Hzの累積Flow差分を50 Hzで集計。ToFの高さでmに換算し、ジャイロで傾きによる見かけの動きを補正。\n姿勢で東・北へ変換して積算。385 count/radは未校正の初期値です。飛行制御には接続しません。
      mask Display: disp('移動距離への換算（表示・記録専用）\n400 Hzの累積Flow差分を50 Hzで集計。ToFの高さでmに換算し、ジャイロで傾きによる見かけの動きを補正。\n姿勢で東・北へ変換して積算。385 count/radは未校正の初期値です。飛行制御には接続しません。')
  MillimetersToMeters : Gain  Gain=single(.001)
  PoseAndRange4 : Mux  Inputs=2
  RangeFields : BusSelector  OutputSignals=DistanceMm
  RangeToSingle : DataTypeConversion  OutDataTypeStr=single  SaturateOnIntegerOverflow=off  RndMeth=Floor
  FlowDistance : Outport
  wires:
  OpticalFlow/1 -> FlowFields/1  "OpticalFlow"
  RangeFields/1 -> RangeToSingle/1  "<DistanceMm>"
  BottomRange/1 -> RangeFields/1  "BottomRange"
  RawIMU/1 -> IMUFields/1  "RawIMU"
  Attitude/1 -> AttitudeFields/1  "Attitude"
  RangeToSingle/1 -> MillimetersToMeters/1
  MillimetersToMeters/1 -> PoseAndRange4/2  "ToFRangeM"
  AttitudeFields/1 -> PoseAndRange4/1  "<Angles>"
  FlowFields/1 -> GroundMotionDistance/1  "<Totals>"
  FlowFields/2 -> GroundMotionDistance/2  "<Raw>"
  IMUFields/1 -> GroundMotionDistance/3  "<AngularRate>"
  PoseAndRange4/1 -> GroundMotionDistance/4  "PoseAndRange"
  GroundMotionDistance/1 -> DistanceData/1  "PositionEN"
  GroundMotionDistance/2 -> DistanceData/2  "Used"
  GroundMotionDistance/3 -> DistanceData/3  "DeltaEN"
  DistanceData/1 -> FlowDistance/1  "FlowDistance"

== system StampFly_KF400/OpticalFlowSensor400 ==
  DeviceRead : MATLABSystem  System=stampfly.PMW3901MB  SampleTime=.0025  SimulateUsing=Code generation
      mask Type: stampfly.PMW3901MB
  JapaneseExplanation : Subsystem  Description=光学フロー取得専用：400 Hz / SPI 2 MHz。生カウント・品質・読出し時間を出力。制御には接続しません。
      mask Display: disp('光学フロー取得専用：400 Hz / SPI 2 MHz。生カウント・品質・読出し時間を出力。制御には接続しません。')
  SensorDataBus : BusCreator  Inputs=4  OutDataTypeStr=Bus: LogFlowBus  NonVirtualBus=on
  OpticalFlow : Outport
  wires:
  DeviceRead/1 -> SensorDataBus/1  "Delta"
  DeviceRead/2 -> SensorDataBus/2  "Raw"
  SensorDataBus/1 -> OpticalFlow/1  "SensorData"
  DeviceRead/3 -> SensorDataBus/3  "Info"
  DeviceRead/4 -> SensorDataBus/4  "Totals"

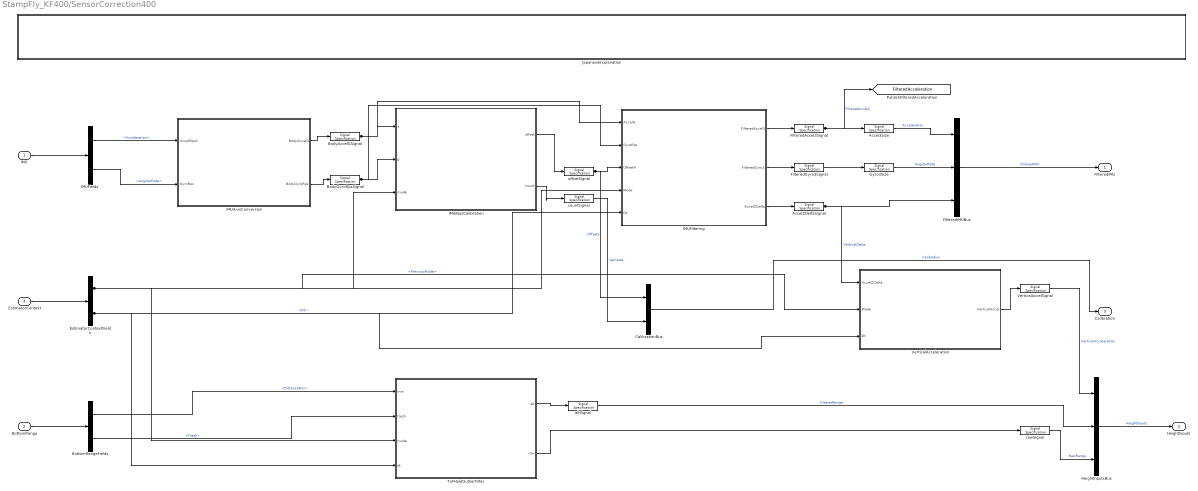
== system StampFly_KF400/SensorCorrection400 ==
  IMU : Inport
  BottomRange : Inport  Port=2
  EstimatorContext : Inport  Port=3
  Accel3Size : SignalSpecification  OutDataTypeStr=single  Dimensions=3
  AccelZDeltaSignal : SignalSpecification  OutDataTypeStr=single  Dimensions=1
  BodyAccelGSignal : SignalSpecification  OutDataTypeStr=single  Dimensions=3
  BodyGyroRpsSignal : SignalSpecification  OutDataTypeStr=single  Dimensions=3
  BottomRangeFields : BusSelector  OutputSignals=DistanceMm,Fresh
  CalibrationBus : BusCreator  Inputs=2
  EstimatorContextFields : BusSelector  OutputSignals=PreviousMode,Dt
  FilteredAccel3Signal : SignalSpecification  OutDataTypeStr=single  Dimensions=3
  FilteredGyro3Signal : SignalSpecification  OutDataTypeStr=single  Dimensions=3
  FilteredIMUBus : BusCreator  Inputs=3
  Gyro3Size : SignalSpecification  OutDataTypeStr=single  Dimensions=3
  HeightInputsBus : BusCreator  Inputs=3
  IMUAxisConversion : Subsystem  Description=BMI270 → 航空機座標
      mask Display: disp('IMUAxisConversion');port_label('input',1,'AccelMps2');port_label('input',2,'GyroRps');port_label('output',1,'BodyAccelG');port_label('output',2,'BodyGyroRps');
  IMUBiasCalibration : MATLAB Function  Description=800サンプルでオフセット推定  TreatAsAtomicUnit=on
  IMUFields : BusSelector  OutputSignals=Acceleration,AngularRate
  IMUFiltering : Subsystem  Description=校正値を引き一次フィルター
      mask Display: disp('IMUFiltering');port_label('input',1,'AccelG');port_label('input',2,'GyroRps');port_label('input',3,'Offset4');port_label('input',4,'Mode');port_label('input',5,'Dt');port_label('output',1,'FilteredAccel3');port_label('output',2,'FilteredGyro3');port_label('output',3,'AccelZDelta');
  JapaneseExplanation : Subsystem  Description=|
      | センサー補正（400 Hz）
      | IMUの軸を機体座標に変換し、800点でバイアスを校正します。
      | 加速度・角速度のフィルターと、下向きToFの最新値保持／外れ値処理を行います。
      | IMU: m/s^2・rad/s → 内部加速度: g。FilteredIMU・HeightInputs・Calibrationへ分けて出力。
      mask Display: disp(sprintf('センサー校正・前処理 / 400 Hz\n機体座標へ変換 → 800点の静止校正 → 加速度・角速度のフィルター\n下向きToFの保持・外れ値処理と鉛直加速度を計算。'));
  ToFHoldOutlierFilter : MATLAB Function  Description=新着距離を判定 / 旧値を保持  TreatAsAtomicUnit=on
  VerticalAccelSignal : SignalSpecification  OutDataTypeStr=single  Dimensions=1
  VerticalAcceleration : Subsystem  Description=重力成分を除去・フィルター
      mask Display: disp('VerticalAcceleration');port_label('input',1,'AccelZDelta');port_label('input',2,'Mode');port_label('input',3,'Dt');port_label('output',1,'VerticalAccel');
  altSignal : SignalSpecification  OutDataTypeStr=single  Dimensions=1
  countSignal : SignalSpecification  OutDataTypeStr=uint16  Dimensions=1
  offsetSignal : SignalSpecification  OutDataTypeStr=single  Dimensions=4
  rawSignal : SignalSpecification  OutDataTypeStr=int16  Dimensions=1
  FilteredIMU : Outport
  HeightInputs : Outport  Port=2
  Calibration : Outport  Port=3
  tag scope: FilteredAcceleration=global
  wires:
  IMU/1 -> IMUFields/1
  IMUFields/1 -> IMUAxisConversion/1(AccelMps2)  "<Acceleration>"
  EstimatorContext/1 -> EstimatorContextFields/1
  IMUAxisConversion/2(BodyGyroRps) -> BodyGyroRpsSignal/1
  IMUFiltering/2(FilteredGyro3) -> FilteredGyro3Signal/1
  BodyAccelGSignal/1 -> IMUFiltering/1(AccelG), IMUBiasCalibration/1(a)
  IMUFields/2 -> IMUAxisConversion/2(GyroRps)  "<AngularRate>"
  IMUAxisConversion/1(BodyAccelG) -> BodyAccelGSignal/1
  BottomRange/1 -> BottomRangeFields/1
  BodyGyroRpsSignal/1 -> IMUFiltering/2(GyroRps), IMUBiasCalibration/2(g)
  EstimatorContextFields/1 -> IMUBiasCalibration/3(mode), IMUFiltering/4(Mode), VerticalAcceleration/2(Mode), ToFHoldOutlierFilter/3(mode)  "<PreviousMode>"
  EstimatorContextFields/2 -> VerticalAcceleration/3(Dt), IMUFiltering/5(Dt), ToFHoldOutlierFilter/4(dt)  "<Dt>"
  BottomRangeFields/1 -> ToFHoldOutlierFilter/1(mm)  "<DistanceMm>"
  BottomRangeFields/2 -> ToFHoldOutlierFilter/2(fresh)  "<Fresh>"
  IMUBiasCalibration/1(offset) -> offsetSignal/1
  IMUBiasCalibration/2(count) -> countSignal/1
  HeightInputsBus/1 -> HeightInputs/1  "HeightInputs"
  ToFHoldOutlierFilter/1(alt) -> altSignal/1
  ToFHoldOutlierFilter/2(raw) -> rawSignal/1
  offsetSignal/1 -> CalibrationBus/1, IMUFiltering/3(Offset4)  "Offsets"
  countSignal/1 -> CalibrationBus/2  "Samples"
  IMUFiltering/1(FilteredAccel3) -> FilteredAccel3Signal/1
  IMUFiltering/3(AccelZDelta) -> AccelZDeltaSignal/1
  CalibrationBus/1 -> Calibration/1  "Calibration"
  rawSignal/1 -> HeightInputsBus/3  "RawRange"
  FilteredAccel3Signal/1 -> [FilteredAcceleration], Accel3Size/1  "FilteredAccelG"
  FilteredGyro3Signal/1 -> Gyro3Size/1
  AccelZDeltaSignal/1 -> FilteredIMUBus/3, VerticalAcceleration/1(AccelZDelta)  "VerticalDelta"
  Accel3Size/1 -> FilteredIMUBus/1  "Acceleration"
  Gyro3Size/1 -> FilteredIMUBus/2  "AngularRate"
  VerticalAcceleration/1(VerticalAccel) -> VerticalAccelSignal/1
  FilteredIMUBus/1 -> FilteredIMU/1  "FilteredIMU"
  altSignal/1 -> HeightInputsBus/2  "FilteredRange"
  VerticalAccelSignal/1 -> HeightInputsBus/1  "VerticalAcceleration"

== system StampFly_KF400/TickStart400 ==
  CycleClock400 : MATLABSystem  Description=GPTimerで400 Hzを起動。実測Dtと時刻、周期診断を出力します。  Priority=1  System=official.TickStart400  SampleTime=Official.Step  SimulateUsing=Code generation
      mask Type: official.TickStart400
  UsToSeconds : Gain  Gain=single(1e-6)  OutDataTypeStr=single
  Dt : Outport
  tag scope: CycleStartUs=global, SamplePeriod=global, SchedulerStatus=global, TimeSeconds=global
  wires:
  CycleClock400/1 -> [CycleStartUs], UsToSeconds/1  "StartUs"
  CycleClock400/2 -> [SamplePeriod], Dt/1
  CycleClock400/3 -> [SchedulerStatus]
  UsToSeconds/1 -> [TimeSeconds]

== system StampFly_KF400/AttitudeAltitudeEstimation400/AltitudeKalman ==
  AltitudeM : Inport
  AccelerationG : Inport  Port=2
  PreviousMode : Inport  Port=3
  Dt : Inport  Port=4
  ParkingReset : Inport  Port=5
  FilterStep : Subsystem  TreatAsAtomicUnit=on
  FlightOutputs : MATLAB Function  TreatAsAtomicUnit=on
  ProcessParameters : Constant  Value=AltitudeKF.ProcessParameters
  UpdateSchedule : MATLAB Function  TreatAsAtomicUnit=on
  HeightM : Outport
  VelocityMps : Outport  Port=2
  EstimatedBias : Outport  Port=3
  wires:
  FlightOutputs/3(bias) -> EstimatedBias/1
  FlightOutputs/2(velocity) -> VelocityMps/1
  FlightOutputs/1(height) -> HeightM/1
  FilterStep/1(StateVector) -> FlightOutputs/1(state)
  UpdateSchedule/1(run) -> FlightOutputs/2(run), FilterStep/Enable  "Run"
  UpdateSchedule/2(filterReset) -> FilterStep/8(Reset)  "CovarianceReset"
  UpdateSchedule/6(Q) -> FilterStep/7(Q)  "ProcessCovariance"
  UpdateSchedule/5(C) -> FilterStep/6(C)  "ObservationMatrix"
  UpdateSchedule/4(B) -> FilterStep/5(B)  "InputMatrix"
  UpdateSchedule/3(A) -> FilterStep/4(A)  "StateMatrix"
  AccelerationG/1 -> FilterStep/2(AccelerationG)
  AltitudeM/1 -> FilterStep/1(AltitudeM)
  ProcessParameters/1 -> UpdateSchedule/4(processParameters), FilterStep/9(ProcessParameters)
  ParkingReset/1 -> UpdateSchedule/3(parkingReset), FlightOutputs/3(parkingReset)
  Dt/1 -> FilterStep/3(Dt), UpdateSchedule/2(dt)
  PreviousMode/1 -> UpdateSchedule/1(mode)

== system StampFly_KF400/AttitudeAltitudeEstimation400/IMUAttitude400 ==
  AngularRate : Inport
  AccelerationG : Inport  Port=2
  PreviousMode : Inport  Port=3
  AttitudeReset : Inport  Port=4
  FilterInputs : MATLAB Function  TreatAsAtomicUnit=on
  FlightOutputs : MATLAB Function  TreatAsAtomicUnit=on
  FusionState : Subsystem  TreatAsAtomicUnit=on
  Angles : Outport
  Quaternion : Outport  Port=2
  CorrectedAngularRate : Outport  Port=3
  wires:
  PreviousMode/1 -> FilterInputs/3(mode)
  AngularRate/1 -> FlightOutputs/5(rawRates), FilterInputs/1(rates)
  AccelerationG/1 -> FilterInputs/2(accelG)
  FilterInputs/4(filterReset) -> FusionState/3(Reset)  "PendingReset"
  AttitudeReset/1 -> FilterInputs/4(reset), FlightOutputs/4(reset)
  FilterInputs/3(run) -> FusionState/Enable, FlightOutputs/3(run)
  FilterInputs/2(gyroRps) -> FusionState/2(Gyro)  "GyroRps"
  FilterInputs/1(accelMps2) -> FusionState/1(Accel)  "AccelMps2"
  FusionState/1(Orientation) -> FlightOutputs/1(orientation)
  FusionState/2(AngularVelocity) -> FlightOutputs/2(angularVelocity)
  FlightOutputs/1(angles) -> Angles/1  "Angles"
  FlightOutputs/2(q) -> Quaternion/1  "Quaternion"
  FlightOutputs/3(rates) -> CorrectedAngularRate/1  "AngularRate"

== system StampFly_KF400/AttitudeAltitudeEstimation400/JapaneseExplanation ==

== system StampFly_KF400/AttitudeAltitudeEstimation400/SensorDiagnosticPack ==
  VerticalAccel : Inport
  KalmanBias : Inport  Port=2
  FilteredRange : Inport  Port=3
  Offsets4 : Inport  Port=4
  Count : Inport  Port=5
  CountToSingle : DataTypeConversion  OutDataTypeStr=single  SaturateOnIntegerOverflow=off  RndMeth=Floor
  PackDiagnostics8 : Mux  Inputs=5
  Diagnostics8 : Outport
  wires:
  CountToSingle/1 -> PackDiagnostics8/5
  Offsets4/1 -> PackDiagnostics8/4
  FilteredRange/1 -> PackDiagnostics8/3
  KalmanBias/1 -> PackDiagnostics8/2
  VerticalAccel/1 -> PackDiagnostics8/1
  Count/1 -> CountToSingle/1
  PackDiagnostics8/1 -> Diagnostics8/1
